simulink subsystem "hys_s"  (R2024b)
settings: Solver=VariableStepAuto  StartTime=0.0  StopTime=10.0  RelTol=1e-3
undefined symbols (not defined in the file): control
settings Model: Creator=pierb  LastModifiedBy=pierb

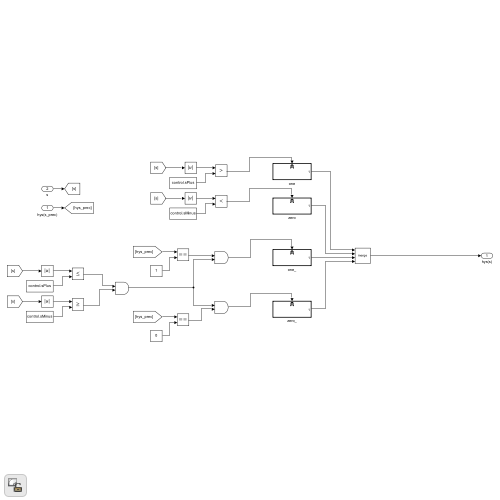
[thumbnail: Simulink's stored preview of the top-level diagram]
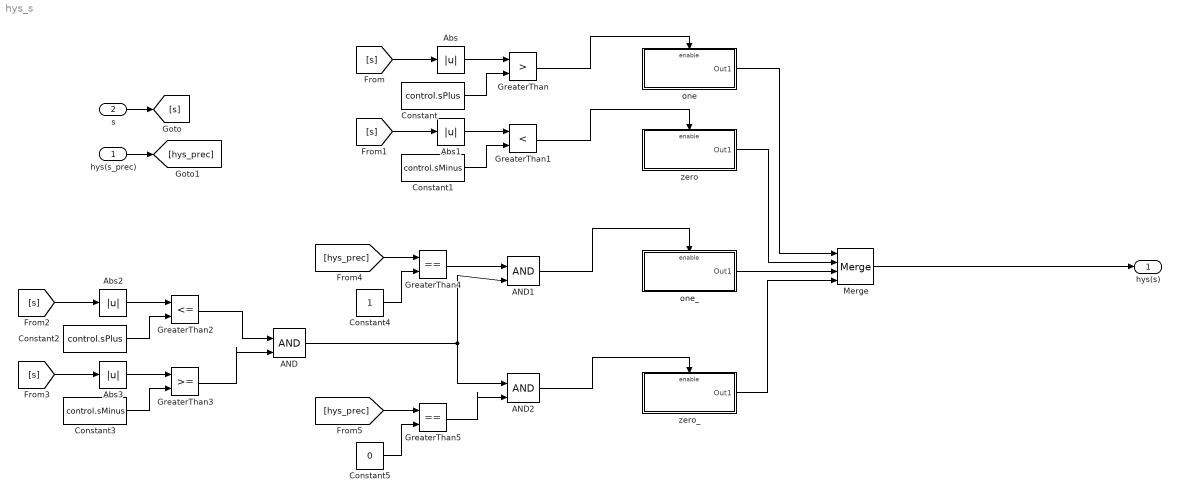
== system hys_s ==
  hys(s_prec) : Inport
  s : Inport  Port=2
  AND : Logic  IconShape=distinctive  AllPortsSameDT=off  OutDataTypeStr=boolean
  AND1 : Logic  IconShape=distinctive  AllPortsSameDT=off  OutDataTypeStr=boolean
  AND2 : Logic  IconShape=distinctive  AllPortsSameDT=off  OutDataTypeStr=boolean
  Abs{,1..3} (4 alike) : Abs  SaturateOnIntegerOverflow=off
  Constant : Constant  Value=control.sPlus
  Constant1 : Constant  Value=control.sMinus
  Constant2 : Constant  Value=control.sPlus
  Constant3 : Constant  Value=control.sMinus
  Constant4 : Constant
  Constant5 : Constant  Value=0
  GreaterThan : RelationalOperator  Operator=>  OutDataTypeStr=boolean  RndMeth=Simplest  InputSameDT=off
  GreaterThan1 : RelationalOperator  Operator=<  OutDataTypeStr=boolean  RndMeth=Simplest  InputSameDT=off
  GreaterThan2 : RelationalOperator  Operator=<=  OutDataTypeStr=boolean  RndMeth=Simplest  InputSameDT=off
  GreaterThan3 : RelationalOperator  OutDataTypeStr=boolean  RndMeth=Simplest  InputSameDT=off
  GreaterThan4 : RelationalOperator  Operator===  OutDataTypeStr=boolean  RndMeth=Simplest  InputSameDT=off
  GreaterThan5 : RelationalOperator  Operator===  OutDataTypeStr=boolean  RndMeth=Simplest  InputSameDT=off
  Merge : Merge  Inputs=4
  one : Subsystem  TreatAsAtomicUnit=on
  one_ : Subsystem  TreatAsAtomicUnit=on
  zero : Subsystem  TreatAsAtomicUnit=on
  zero_ : Subsystem  TreatAsAtomicUnit=on
  hys(s) : Outport
  wires:
  Abs/1 -> GreaterThan/1
  Constant/1 -> GreaterThan/2
  s/1 -> [s]
  [s] -> Abs/1
  GreaterThan/1 -> one/Enable
  GreaterThan1/1 -> zero/Enable
  [s] -> Abs1/1
  Constant1/1 -> GreaterThan1/2
  Abs1/1 -> GreaterThan1/1
  [s] -> Abs2/1
  Abs2/1 -> GreaterThan2/1
  Constant2/1 -> GreaterThan2/2
  GreaterThan2/1 -> AND/1
  Constant3/1 -> GreaterThan3/2
  Abs3/1 -> GreaterThan3/1
  [s] -> Abs3/1
  GreaterThan3/1 -> AND/2
  AND/1 -> AND2/1, AND1/2
  hys(s_prec)/1 -> [hys_prec]
  GreaterThan4/1 -> AND1/1
  [hys_prec] -> GreaterThan4/1
  Constant4/1 -> GreaterThan4/2
  Constant5/1 -> GreaterThan5/2
  [hys_prec] -> GreaterThan5/1
  GreaterThan5/1 -> AND2/2
  AND1/1 -> one_/Enable
  AND2/1 -> zero_/Enable
  one/1(Out1) -> Merge/1
  zero/1(Out1) -> Merge/2
  one_/1(Out1) -> Merge/3
  zero_/1(Out1) -> Merge/4
  Merge/1 -> hys(s)/1

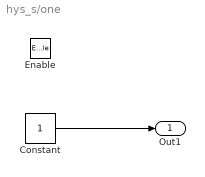
== system hys_s/one ==
  Enable : EnablePort
  Constant : Constant
  Out1 : Outport
  wires:
  Constant/1 -> Out1/1

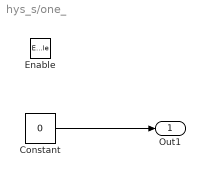
== system hys_s/one_ ==
  Enable : EnablePort
  Constant : Constant  Value=0
  Out1 : Outport
  wires:
  Constant/1 -> Out1/1

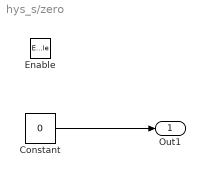
== system hys_s/zero ==
  Enable : EnablePort
  Constant : Constant  Value=0
  Out1 : Outport
  wires:
  Constant/1 -> Out1/1

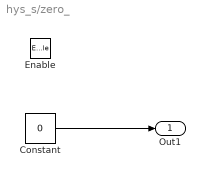
== system hys_s/zero_ ==
  Enable : EnablePort
  Constant : Constant  Value=0
  Out1 : Outport
  wires:
  Constant/1 -> Out1/1
